simulink model "Landing_Gear_Subsystem"  (R2026b)
settings: Solver=VariableStepAuto
settings Model: Creator=Teama  LastModifiedBy=Teama

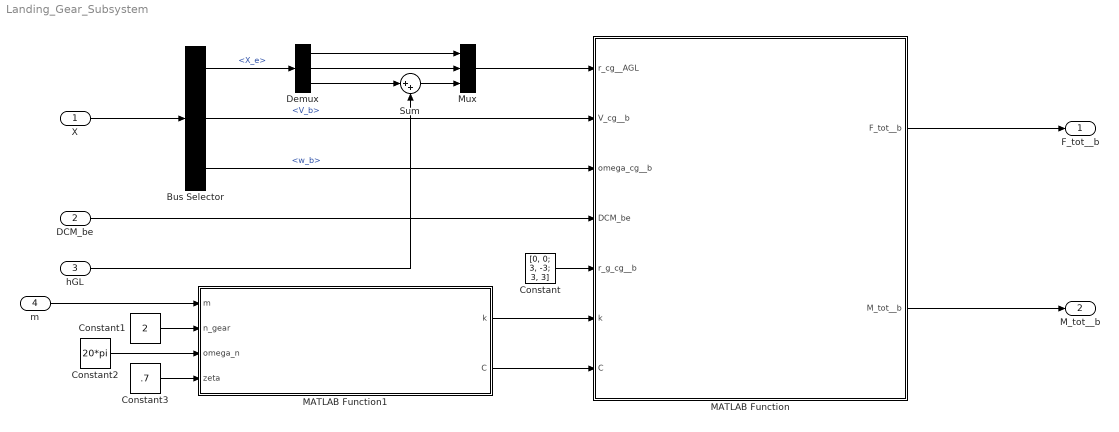
== system Landing_Gear_Subsystem ==
  X : Inport
  DCM_be : Inport  Port=2
  hGL : Inport  Port=3
  m : Inport  Port=4
  Bus Selector : BusSelector  OutputSignals=X_e,V_b,w_b
  Constant : Constant  Value=[0, 0; 3, -3; 3, 3]
  Constant1 : Constant  Value=2
  Constant2 : Constant  Value=20*pi
  Constant3 : Constant  Value=.7
  Demux : Demux  Outputs=3
  MATLAB Function : MATLAB Function  TreatAsAtomicUnit=on
  MATLAB Function1 : MATLAB Function  TreatAsAtomicUnit=on
  Mux : Mux  Inputs=3
  Sum : Sum  Inputs=|++
  F_tot__b : Outport
  M_tot__b : Outport  Port=2
  wires:
  MATLAB Function/2(M_tot__b) -> M_tot__b/1
  MATLAB Function/1(F_tot__b) -> F_tot__b/1
  X/1 -> Bus Selector/1
  Bus Selector/1 -> Demux/1  "<X_e>"
  Demux/3 -> Sum/1
  hGL/1 -> Sum/2
  Sum/1 -> Mux/3
  Demux/2 -> Mux/2
  Demux/1 -> Mux/1
  Mux/1 -> MATLAB Function/1(r_cg__AGL)
  Bus Selector/2 -> MATLAB Function/2(V_cg__b)  "<V_b>"
  Bus Selector/3 -> MATLAB Function/3(omega_cg__b)  "<w_b>"
  DCM_be/1 -> MATLAB Function/4(DCM_be)
  Constant/1 -> MATLAB Function/5(r_g_cg__b)
  MATLAB Function1/1(k) -> MATLAB Function/6(k)
  MATLAB Function1/2(C) -> MATLAB Function/7(C)
  m/1 -> MATLAB Function1/1(m)
  Constant1/1 -> MATLAB Function1/2(n_gear)
  Constant2/1 -> MATLAB Function1/3(omega_n)
  Constant3/1 -> MATLAB Function1/4(zeta)

== matlab function Landing_Gear_Subsystem/MATLAB Function ==
  data: F_tot__b output double size=[3,1]; M_tot__b output double size=[3,1]; r_cg__AGL input; V_cg__b input; omega_cg__b input; DCM_be input; r_g_cg__b input; k input; C input
function [F_tot__b, M_tot__b] = landing_gear_wrapper(r_cg__AGL, V_cg__b, omega_cg__b, DCM_be, r_g_cg__b, k, C)
    % each landing gear r_g_cg__b is in the columns of r_g_cg__b
    F_tot__b = zeros(3,1);
    M_tot__b = zeros(3,1);
    
    [F1_tot__b, M1_tot__b] = landing_gear(r_cg__AGL, V_cg__b, omega_cg__b, DCM_be, r_g_cg__b(:,1), k, C);
    [F2_tot__b, M2_tot__b] = landing_gear(r_cg__AGL, V_cg__b, omega_cg__b, DCM_be, r_g_cg__b(:,2), k, C);

    F_tot__b = F1_tot__b + F2_tot__b;
    M_tot__b = M1_tot__b + M2_tot__b;
end

== matlab function Landing_Gear_Subsystem/MATLAB Function1 ==
  data: m input; k output; n_gear input; omega_n input; zeta input; C output
function [k, C] = gear_parameterization_wrapper(m, n_gear, omega_n, zeta)
    k = 0;
    C = 0;

    [k, C] = gear_parameterization(m, n_gear, omega_n, zeta);
end
